simulink model "CabinTempController"  (R2015a)
settings: Solver=FixedStepDiscrete  StartTime=0.0  StopTime=10.0  FixedStep=0.01  RelTol=1e-3
libraries: simulink x2
settings Model: Creator=A.hegazy  LastModifiedBy=A.hegazy
settings DataIOCC: SaveFormat=Dataset
settings OptimizationCC: OptimizeModelRefInitCode=on  LifeSpan=1
settings HardwareCC: ProdBitPerPointer=64  ProdLongLongMode=on  ProdHWDeviceType=Generic->64-bit Embedded Processor (LLP64)  TargetBitPerLong=64  TargetBitPerPointer=64  TargetIntDivRoundTo=Zero  TargetEndianess=LittleEndian  TargetWordSize=64  TargetHWDeviceType=Intel->x86-64
settings RTWCC: SystemTargetFile=ert.tlc  TemplateMakefile=ert_default_tmf  Description=Embedded Coder  GenerateReport=on  PortableWordSizes=on  CreateSILPILBlock=SIL
settings CodeAppCC: IgnoreCustomStorageClasses=off
settings ERTTargetCC: ParMdlRefBuildCompliant=on  CompOptLevelCompliant=on  ConcurrentExecutionCompliant=on  ERTFirstTimeCompliant=on  SupportContinuousTime=off  SupportVariableSizeSignals=off  ModelStepFunctionPrototypeControlCompliant=on  CPPClassGenCompliant=on  InlinedParameterPlacement=Hierarchical  ERTCustomFileTemplate=example_file_process.tlc

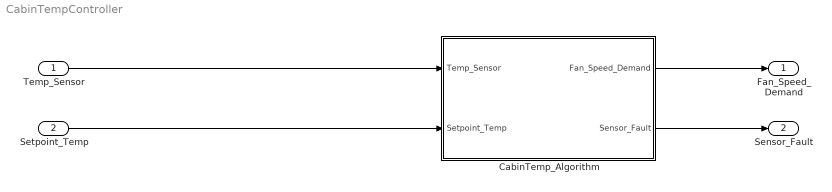
== system CabinTempController ==
  Temp_Sensor : Inport
  Setpoint_Temp : Inport  Port=2
  CabinTemp_Algorithm : Subsystem  TreatAsAtomicUnit=on  SystemSampleTime=0.01
  Fan_Speed_Demand : Outport
  Sensor_Fault : Outport  Port=2
  wires:
  Temp_Sensor/1 -> CabinTemp_Algorithm/1(Temp_Sensor)
  Setpoint_Temp/1 -> CabinTemp_Algorithm/2(Setpoint_Temp)
  CabinTemp_Algorithm/1(Fan_Speed_Demand) -> Fan_Speed_Demand/1
  CabinTemp_Algorithm/2(Sensor_Fault) -> Sensor_Fault/1

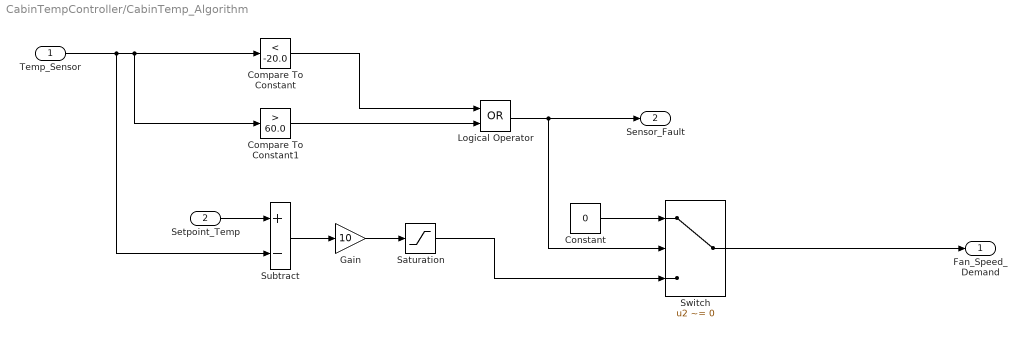
== system CabinTempController/CabinTemp_Algorithm ==
  Temp_Sensor : Inport  OutDataTypeStr=single  SampleTime=0.01
  Setpoint_Temp : Inport  Port=2  OutDataTypeStr=single  SampleTime=0.01
  Compare To Constant : simulink/Logic and Bit Operations/Compare To Constant  relop=<  const=-20.0  OutDataTypeStr=boolean
  Compare To Constant1 : simulink/Logic and Bit Operations/Compare To Constant  relop=>  const=60.0  OutDataTypeStr=boolean
  Constant : Constant  Value=0  OutDataTypeStr=single
  Gain : Gain  Gain=10
  Logical Operator : Logic  Operator=OR  AllPortsSameDT=off  OutDataTypeStr=boolean
  Saturation : Saturate  UpperLimit=100  LowerLimit=0
  Subtract : Sum  Inputs=+-
  Switch : Switch  Criteria=u2 ~= 0
  Fan_Speed_Demand : Outport  OutDataTypeStr=single
  Sensor_Fault : Outport  Port=2  OutDataTypeStr=boolean
  wires:
  Temp_Sensor/1 -> Subtract/2, Compare To Constant1/1, Compare To Constant/1
  Compare To Constant/1 -> Logical Operator/1
  Compare To Constant1/1 -> Logical Operator/2
  Logical Operator/1 -> Switch/2, Sensor_Fault/1
  Setpoint_Temp/1 -> Subtract/1
  Subtract/1 -> Gain/1
  Gain/1 -> Saturation/1
  Constant/1 -> Switch/1
  Saturation/1 -> Switch/3
  Switch/1 -> Fan_Speed_Demand/1
